simulink model "huffman_ext"  (R2023b)
settings: Solver=FixedStepDiscrete  StartTime=0.0  StopTime=(Nbits-1)*Tb  FixedStep=Tb  RelTol=1e-3
undefined symbols (not defined in the file): graine, kk, p1_ext, poids, tab_long, Tb
settings Model: Creator=e2507457  LastModifiedBy=e2507457

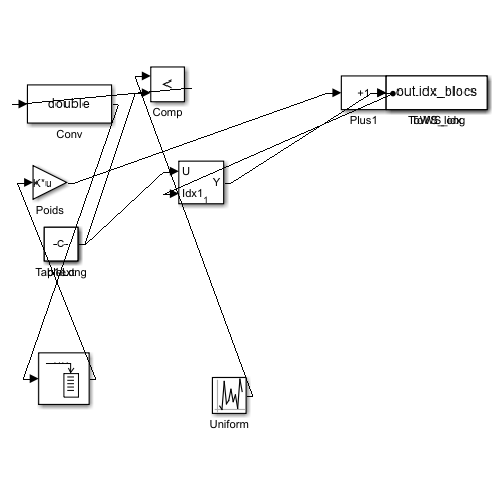
[thumbnail: Simulink's stored preview of the top-level diagram]
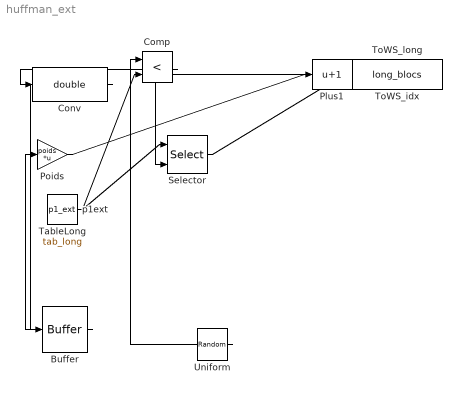
== system huffman_ext ==
  Buffer : Buffer  N=kk
  Comp : RelationalOperator  Operator=<  OutDataTypeStr=boolean  RndMeth=Simplest  InputSameDT=off
  Conv : DataTypeConversion  OutDataTypeStr=double  SaturateOnIntegerOverflow=off  RndMeth=Floor
  Plus1 : Bias  Bias=1  SaturateOnIntegerOverflow=off
  Poids : Gain  Gain=poids  Multiplication=Matrix(K*u)
  Selector : Selector  InputPortWidth=2^kk  IndexOptions=Index vector (port)  Indices=[1 3]  OutputSizes=1
  TableLong : Constant  Value=tab_long
  ToWS_idx : ToWorkspace  VariableName=idx_blocs  SampleTime=-1
  ToWS_long : ToWorkspace  VariableName=long_blocs  SampleTime=-1
  Uniform : UniformRandomNumber  Minimum=0  Seed=graine  SampleTime=Tb
  p1ext : Constant  Value=p1_ext  SampleTime=Tb
  wires:
  Uniform/1 -> Comp/1
  p1ext/1 -> Comp/2
  Comp/1 -> Conv/1
  Conv/1 -> Buffer/1
  Buffer/1 -> Poids/1
  Poids/1 -> Plus1/1
  Plus1/1 -> Selector/2, ToWS_idx/1
  TableLong/1 -> Selector/1
  Selector/1 -> ToWS_long/1
